simulink model "ps_isop_rail"  (R2026a)
settings: Solver=ode23tb  StopTime=param.sim.simlength  FixedStep=param.glb_time.tc  MaxStep=param.glb_time.tc
values from neighbouring files (symbols this model uses):
  param = struct()    [init_model.m]
libraries: fl_lib x49, nesl_utility x38, full_bridge_ideal_switch x4, single_phase_transformer x4, pi_ctrl x3, full_bridge_diode_rectifier x2, lithium_ion_battery x1, full_bridge_zvs_pwm_modulator x1, discrete_time_low_pass_filter x1
(part 2 of 2)

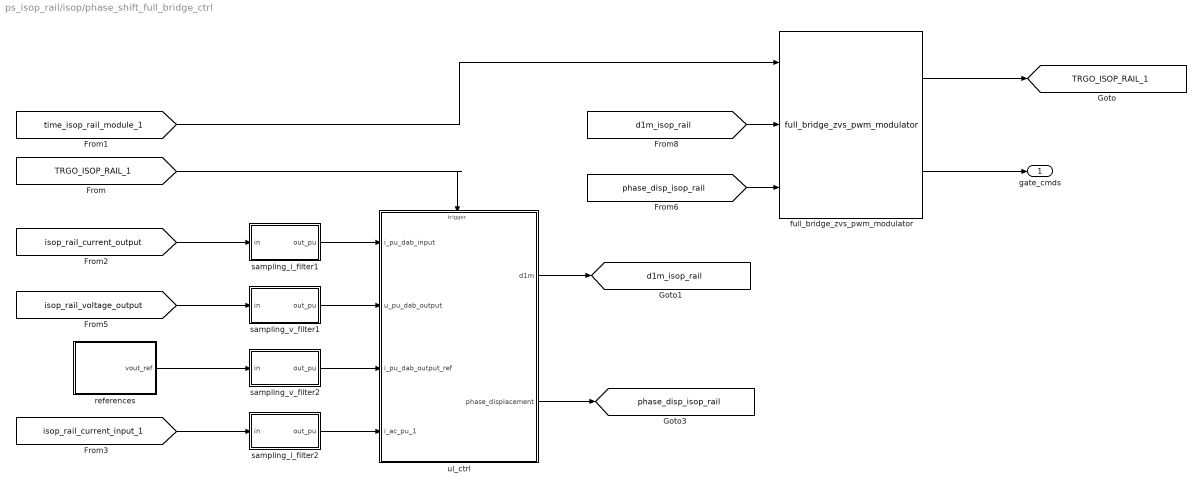
== system ps_isop_rail/isop/phase_shift_full_bridge_ctrl ==
  full_bridge_zvs_pwm_modulator : full_bridge_zvs_pwm_modulator/full_bridge_zvs_pwm_modulator  fPWM_m=param.glb_time.fPWM_ISOP_RAIL  m_up_m=1  m_low_m=0  dead_time_DAB_m=param.glb_time.dead_time_ISOP_RAIL  pos_cmd_gate_m=15  neg_cmd_gate_m=-10  polarity_m=1  tc_m=param.glb_time.tc  max_phase_displacement_m=pi  trgo_double_update_m=param.glb_time.TRGO_ISOP_RAIL_double_update
  references : Subsystem
  sampling_i_filter1 : Subsystem
  sampling_i_filter2 : Subsystem
  sampling_v_filter1 : Subsystem
  sampling_v_filter2 : Subsystem
  ui_ctrl : Subsystem
  gate_cmds : Outport
  tag scope: TRGO_ISOP_RAIL_1=global, d1m_isop_rail=global, phase_disp_isop_rail=global
  wires:
  [isop_rail_voltage_output] -> sampling_v_filter1/1(in)
  [isop_rail_current_output] -> sampling_i_filter1/1(in)
  sampling_i_filter1/1(out_pu) -> ui_ctrl/1(i_pu_dab_input)
  sampling_v_filter1/1(out_pu) -> ui_ctrl/2(u_pu_dab_output)
  sampling_v_filter2/1(out_pu) -> ui_ctrl/3(i_pu_dab_output_ref)
  references/1(vout_ref) -> sampling_v_filter2/1(in)
  full_bridge_zvs_pwm_modulator/2 -> gate_cmds/1
  [time_isop_rail_module_1] -> full_bridge_zvs_pwm_modulator/1
  full_bridge_zvs_pwm_modulator/1 -> [TRGO_ISOP_RAIL_1]
  [TRGO_ISOP_RAIL_1] -> ui_ctrl/Trigger
  [isop_rail_current_input_1] -> sampling_i_filter2/1(in)
  sampling_i_filter2/1(out_pu) -> ui_ctrl/4(i_ac_pu_1)
  ui_ctrl/1(d1m) -> [d1m_isop_rail]
  ui_ctrl/2(phase_displacement) -> [phase_disp_isop_rail]
  [phase_disp_isop_rail] -> full_bridge_zvs_pwm_modulator/3
  [d1m_isop_rail] -> full_bridge_zvs_pwm_modulator/2

== system ps_isop_rail/isop/rectifier_1 ==
  full_bridge_diode_rectifier : full_bridge_diode_rectifier/full_bridge_diode_rectifier  Vf_diode_rectifier=param.diode.rectifier.Vf  Rdon_diode_rectifier=param.diode.rectifier.Rdon  Csnubber=param.diode.rectifier.Csnubber  Rsnubber=param.diode.rectifier.Rsnubber
  uac_2(+) : PMIOPort  Side=Left
  uac_2(-) : PMIOPort  Port=2  Side=Left
  udc_1(+) : PMIOPort  Port=3  Side=Right
  udc_1(-) : PMIOPort  Port=4  Side=Right
  tag scope: diode_bridge_1=global
  wires:
  full_bridge_diode_rectifier/1 -> [diode_bridge_1]
  connections:
  udc_1(-)/RConn1 -- full_bridge_diode_rectifier/RConn2
  full_bridge_diode_rectifier/LConn1 -- uac_2(+)/RConn1
  full_bridge_diode_rectifier/LConn2 -- uac_2(-)/RConn1
  udc_1(+)/RConn1 -- full_bridge_diode_rectifier/RConn1

== system ps_isop_rail/isop/rectifier_2 ==
  full_bridge_diode_rectifier : full_bridge_diode_rectifier/full_bridge_diode_rectifier  Vf_diode_rectifier=param.diode.rectifier.Vf  Rdon_diode_rectifier=param.diode.rectifier.Rdon  Csnubber=param.diode.rectifier.Csnubber  Rsnubber=param.diode.rectifier.Rsnubber
  uac_2(+) : PMIOPort  Side=Left
  uac_2(-) : PMIOPort  Port=2  Side=Left
  udc_2(+) : PMIOPort  Port=3  Side=Right
  udc_2(-) : PMIOPort  Port=4  Side=Right
  tag scope: diode_bridge_2=global
  wires:
  full_bridge_diode_rectifier/1 -> [diode_bridge_2]
  connections:
  udc_2(+)/RConn1 -- full_bridge_diode_rectifier/RConn1
  full_bridge_diode_rectifier/LConn2 -- uac_2(-)/RConn1
  full_bridge_diode_rectifier/LConn1 -- uac_2(+)/RConn1
  udc_2(-)/RConn1 -- full_bridge_diode_rectifier/RConn2

== system ps_isop_rail/isop/fb_iso_mod_1/full_bridge ==
  gate_commands : Inport
  full-bridge_ideal_switch_based : Subsystem
  uac_1(+) : PMIOPort  Side=Left
  uac_1(-) : PMIOPort  Port=2  Side=Left
  Udc(+) : PMIOPort  Port=3  Side=Right
  Udc(-) : PMIOPort  Port=4  Side=Right
  wires:
  gate_commands/1 -> full-bridge_ideal_switch_based/1(gate_commands)
  connections:
  uac_1(-)/RConn1 -- full-bridge_ideal_switch_based/RConn2
  Udc(-)/RConn1 -- full-bridge_ideal_switch_based/LConn2
  Udc(+)/RConn1 -- full-bridge_ideal_switch_based/LConn1
  full-bridge_ideal_switch_based/RConn1 -- uac_1(+)/RConn1

== system ps_isop_rail/isop/fb_iso_mod_1/transformers ==
  Current Sensor1 : fl_lib/Electrical/Electrical Sensors/Current Sensor
  Voltage Sensor1 : fl_lib/Electrical/Electrical Sensors/Voltage Sensor
  i1_transformer : nesl_utility/PS-Simulink Converter  PhysicalDomain=network_engine_domain  SubClassName=ps_output  LeftPortType=input  RightPortType=output  PseudoPeriodic=off  Frequencies=[]  VectorFormat=1-D array  Unit=A  AffineConversion=off
  trafo_1 : Subsystem
  u1_transformer : nesl_utility/PS-Simulink Converter  PhysicalDomain=network_engine_domain  SubClassName=ps_output  LeftPortType=input  RightPortType=output  PseudoPeriodic=off  Frequencies=[]  VectorFormat=1-D array  Unit=V  AffineConversion=on
  uac_1(+) : PMIOPort  Side=Left
  uac_1(-) : PMIOPort  Port=2  Side=Left
  uac_2(+) : PMIOPort  Port=3  Side=Right
  uac_2(-) : PMIOPort  Port=4  Side=Right
  tag scope: i1_trafo_mod_1=global, u1_trafo_mod_1=global
  wires:
  u1_transformer/1 -> [u1_trafo_mod_1]
  i1_transformer/1 -> [i1_trafo_mod_1]
  connections:
  trafo_1/LConn1 -- Current Sensor1/RConn2
  uac_1(-)/RConn1 -- Voltage Sensor1/RConn2 -- trafo_1/LConn2
  trafo_1/RConn1 -- uac_2(+)/RConn1
  trafo_1/RConn2 -- uac_2(-)/RConn1
  Voltage Sensor1/LConn1 -- Current Sensor1/LConn1 -- uac_1(+)/RConn1
  Voltage Sensor1/RConn1 -- u1_transformer/LConn1
  Current Sensor1/RConn1 -- i1_transformer/LConn1

== system ps_isop_rail/isop/fb_iso_mod_2/full_bridge ==
  gate_commands : Inport
  full-bridge_ideal_switch_based : Subsystem
  uac_1(+) : PMIOPort  Side=Left
  uac_1(-) : PMIOPort  Port=2  Side=Left
  Udc(+) : PMIOPort  Port=3  Side=Right
  Udc(-) : PMIOPort  Port=4  Side=Right
  wires:
  gate_commands/1 -> full-bridge_ideal_switch_based/1(gate_commands)
  connections:
  full-bridge_ideal_switch_based/RConn1 -- uac_1(+)/RConn1
  Udc(+)/RConn1 -- full-bridge_ideal_switch_based/LConn1
  Udc(-)/RConn1 -- full-bridge_ideal_switch_based/LConn2
  uac_1(-)/RConn1 -- full-bridge_ideal_switch_based/RConn2

== system ps_isop_rail/isop/fb_iso_mod_2/transformers ==
  Current Sensor1 : fl_lib/Electrical/Electrical Sensors/Current Sensor
  Voltage Sensor1 : fl_lib/Electrical/Electrical Sensors/Voltage Sensor
  i1_transformer : nesl_utility/PS-Simulink Converter  PhysicalDomain=network_engine_domain  SubClassName=ps_output  LeftPortType=input  RightPortType=output  PseudoPeriodic=off  Frequencies=[]  VectorFormat=1-D array  Unit=A  AffineConversion=off
  trafo_1 : Subsystem
  u1_transformer : nesl_utility/PS-Simulink Converter  PhysicalDomain=network_engine_domain  SubClassName=ps_output  LeftPortType=input  RightPortType=output  PseudoPeriodic=off  Frequencies=[]  VectorFormat=1-D array  Unit=V  AffineConversion=on
  uac_1(+) : PMIOPort  Side=Left
  uac_1(-) : PMIOPort  Port=2  Side=Left
  uac_2(+) : PMIOPort  Port=3  Side=Right
  uac_2(-) : PMIOPort  Port=4  Side=Right
  tag scope: i1_trafo_mod_2=global, u1_trafo_mod_2=global
  wires:
  i1_transformer/1 -> [i1_trafo_mod_2]
  u1_transformer/1 -> [u1_trafo_mod_2]
  connections:
  Current Sensor1/RConn1 -- i1_transformer/LConn1
  Voltage Sensor1/RConn1 -- u1_transformer/LConn1
  uac_1(+)/RConn1 -- Current Sensor1/LConn1 -- Voltage Sensor1/LConn1
  trafo_1/RConn2 -- uac_2(-)/RConn1
  trafo_1/RConn1 -- uac_2(+)/RConn1
  trafo_1/LConn2 -- Voltage Sensor1/RConn2 -- uac_1(-)/RConn1
  trafo_1/LConn1 -- Current Sensor1/RConn2

== system ps_isop_rail/isop/fb_iso_mod_3/full_bridge ==
  gate_commands : Inport
  full-bridge_ideal_switch_based : Subsystem
  uac_1(+) : PMIOPort  Side=Left
  uac_1(-) : PMIOPort  Port=2  Side=Left
  Udc(+) : PMIOPort  Port=3  Side=Right
  Udc(-) : PMIOPort  Port=4  Side=Right
  wires:
  gate_commands/1 -> full-bridge_ideal_switch_based/1(gate_commands)
  connections:
  uac_1(-)/RConn1 -- full-bridge_ideal_switch_based/RConn2
  Udc(-)/RConn1 -- full-bridge_ideal_switch_based/LConn2
  Udc(+)/RConn1 -- full-bridge_ideal_switch_based/LConn1
  full-bridge_ideal_switch_based/RConn1 -- uac_1(+)/RConn1

== system ps_isop_rail/isop/fb_iso_mod_3/transformers ==
  Current Sensor1 : fl_lib/Electrical/Electrical Sensors/Current Sensor
  Voltage Sensor1 : fl_lib/Electrical/Electrical Sensors/Voltage Sensor
  i1_transformer : nesl_utility/PS-Simulink Converter  PhysicalDomain=network_engine_domain  SubClassName=ps_output  LeftPortType=input  RightPortType=output  PseudoPeriodic=off  Frequencies=[]  VectorFormat=1-D array  Unit=A  AffineConversion=off
  trafo_1 : Subsystem
  u1_transformer : nesl_utility/PS-Simulink Converter  PhysicalDomain=network_engine_domain  SubClassName=ps_output  LeftPortType=input  RightPortType=output  PseudoPeriodic=off  Frequencies=[]  VectorFormat=1-D array  Unit=V  AffineConversion=on
  uac_1(+) : PMIOPort  Side=Left
  uac_1(-) : PMIOPort  Port=2  Side=Left
  uac_2(+) : PMIOPort  Port=3  Side=Right
  uac_2(-) : PMIOPort  Port=4  Side=Right
  tag scope: i1_trafo_mod_3=global, u1_trafo_mod_3=global
  wires:
  u1_transformer/1 -> [u1_trafo_mod_3]
  i1_transformer/1 -> [i1_trafo_mod_3]
  connections:
  trafo_1/LConn1 -- Current Sensor1/RConn2
  uac_1(-)/RConn1 -- Voltage Sensor1/RConn2 -- trafo_1/LConn2
  trafo_1/RConn1 -- uac_2(+)/RConn1
  trafo_1/RConn2 -- uac_2(-)/RConn1
  Voltage Sensor1/LConn1 -- Current Sensor1/LConn1 -- uac_1(+)/RConn1
  Voltage Sensor1/RConn1 -- u1_transformer/LConn1
  Current Sensor1/RConn1 -- i1_transformer/LConn1

== system ps_isop_rail/isop/fb_iso_mod_4/full_bridge ==
  gate_commands : Inport
  full-bridge_ideal_switch_based : Subsystem
  uac_1(+) : PMIOPort  Side=Left
  uac_1(-) : PMIOPort  Port=2  Side=Left
  Udc(+) : PMIOPort  Port=3  Side=Right
  Udc(-) : PMIOPort  Port=4  Side=Right
  wires:
  gate_commands/1 -> full-bridge_ideal_switch_based/1(gate_commands)
  connections:
  full-bridge_ideal_switch_based/RConn1 -- uac_1(+)/RConn1
  Udc(+)/RConn1 -- full-bridge_ideal_switch_based/LConn1
  Udc(-)/RConn1 -- full-bridge_ideal_switch_based/LConn2
  uac_1(-)/RConn1 -- full-bridge_ideal_switch_based/RConn2

== system ps_isop_rail/isop/fb_iso_mod_4/transformers ==
  Current Sensor1 : fl_lib/Electrical/Electrical Sensors/Current Sensor
  Voltage Sensor1 : fl_lib/Electrical/Electrical Sensors/Voltage Sensor
  i1_transformer : nesl_utility/PS-Simulink Converter  PhysicalDomain=network_engine_domain  SubClassName=ps_output  LeftPortType=input  RightPortType=output  PseudoPeriodic=off  Frequencies=[]  VectorFormat=1-D array  Unit=A  AffineConversion=off
  trafo_1 : Subsystem
  u1_transformer : nesl_utility/PS-Simulink Converter  PhysicalDomain=network_engine_domain  SubClassName=ps_output  LeftPortType=input  RightPortType=output  PseudoPeriodic=off  Frequencies=[]  VectorFormat=1-D array  Unit=V  AffineConversion=on
  uac_1(+) : PMIOPort  Side=Left
  uac_1(-) : PMIOPort  Port=2  Side=Left
  uac_2(+) : PMIOPort  Port=3  Side=Right
  uac_2(-) : PMIOPort  Port=4  Side=Right
  tag scope: i1_trafo_mod_4=global, u1_trafo_mod_4=global
  wires:
  i1_transformer/1 -> [i1_trafo_mod_4]
  u1_transformer/1 -> [u1_trafo_mod_4]
  connections:
  Current Sensor1/RConn1 -- i1_transformer/LConn1
  Voltage Sensor1/RConn1 -- u1_transformer/LConn1
  uac_1(+)/RConn1 -- Current Sensor1/LConn1 -- Voltage Sensor1/LConn1
  trafo_1/RConn2 -- uac_2(-)/RConn1
  trafo_1/RConn1 -- uac_2(+)/RConn1
  trafo_1/LConn2 -- Voltage Sensor1/RConn2 -- uac_1(-)/RConn1
  trafo_1/LConn1 -- Current Sensor1/RConn2

== system ps_isop_rail/isop/phase_shift_full_bridge_ctrl/references ==
  Rate Limiter : RateLimiter  RisingSlewLimit=param.isop_rail.hw.idc2_nom*10  FallingSlewLimit=-param.isop_rail.hw.idc2_nom*10  SampleTimeMode=inherited
  Vout_dc_nom : Step  Time=0.025  FinalValue=param.isop_rail.hw.idc2_nom  SampleTime=0
  vout_ref : Outport
  wires:
  Rate Limiter/1 -> vout_ref/1
  Vout_dc_nom/1 -> Rate Limiter/1

== system ps_isop_rail/isop/phase_shift_full_bridge_ctrl/sampling_i_filter1 ==
  in : Inport
  1/Ti3 : Gain  Gain=1/param.isop_rail.hw.idc2_bez  OutDataTypeStr=double  SaturateOnIntegerOverflow=on  ParamDataTypeStr=Inherit: Same as input
  out_pu : Outport
  wires:
  in/1 -> 1/Ti3/1
  1/Ti3/1 -> out_pu/1

== system ps_isop_rail/isop/phase_shift_full_bridge_ctrl/sampling_i_filter2 ==
  in : Inport
  1/Ti3 : Gain  Gain=1/param.isop_rail.hw.idc1_bez  OutDataTypeStr=double  SaturateOnIntegerOverflow=on  ParamDataTypeStr=Inherit: Same as input
  out_pu : Outport
  wires:
  1/Ti3/1 -> out_pu/1
  in/1 -> 1/Ti3/1

== system ps_isop_rail/isop/phase_shift_full_bridge_ctrl/sampling_v_filter1 ==
  in : Inport
  1/Ti3 : Gain  Gain=1/param.isop_rail.hw.udc2_bez  OutDataTypeStr=double  SaturateOnIntegerOverflow=on  ParamDataTypeStr=Inherit: Same as input
  out_pu : Outport
  wires:
  in/1 -> 1/Ti3/1
  1/Ti3/1 -> out_pu/1

== system ps_isop_rail/isop/phase_shift_full_bridge_ctrl/sampling_v_filter2 ==
  in : Inport
  1/Ti3 : Gain  Gain=1/param.isop_rail.hw.idc2_nom  OutDataTypeStr=double  SaturateOnIntegerOverflow=on  ParamDataTypeStr=Inherit: Same as input
  Saturation : Saturate  UpperLimit=1  LowerLimit=0  OutDataTypeStr=double
  out_pu : Outport
  wires:
  in/1 -> 1/Ti3/1
  1/Ti3/1 -> Saturation/1
  Saturation/1 -> out_pu/1

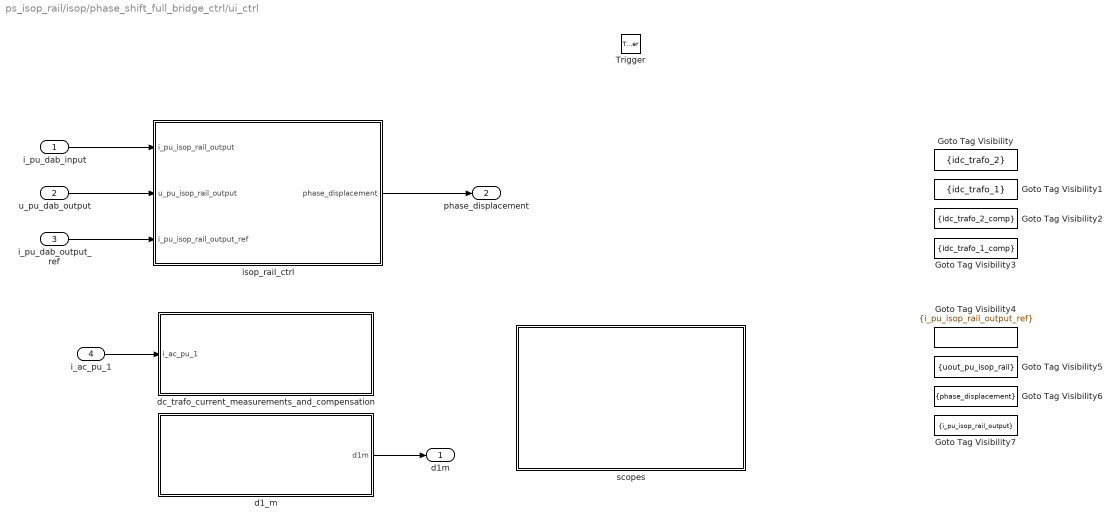
== system ps_isop_rail/isop/phase_shift_full_bridge_ctrl/ui_ctrl ==
  i_pu_dab_input : Inport
  u_pu_dab_output : Inport  Port=2
  i_pu_dab_output_ref : Inport  Port=3
  i_ac_pu_1 : Inport  Port=4
  Trigger : TriggerPort  VariantControl=(inherit)  PortDimensions=1
  Goto Tag Visibility : GotoTagVisibility  GotoTag=idc_trafo_2
  Goto Tag Visibility1 : GotoTagVisibility  GotoTag=idc_trafo_1
  Goto Tag Visibility2 : GotoTagVisibility  GotoTag=idc_trafo_2_comp
  Goto Tag Visibility3 : GotoTagVisibility  GotoTag=idc_trafo_1_comp
  Goto Tag Visibility4 : GotoTagVisibility  GotoTag=i_pu_isop_rail_output_ref
  Goto Tag Visibility5 : GotoTagVisibility  GotoTag=uout_pu_isop_rail
  Goto Tag Visibility6 : GotoTagVisibility  GotoTag=phase_displacement
  Goto Tag Visibility7 : GotoTagVisibility  GotoTag=i_pu_isop_rail_output
  d1_m : Subsystem
  dc_trafo_current_measurements_and_compensation : Subsystem
  isop_rail_ctrl : Subsystem
  scopes : Subsystem
  d1m : Outport
  phase_displacement : Outport  Port=2
  wires:
  i_pu_dab_input/1 -> isop_rail_ctrl/1(i_pu_isop_rail_output)
  u_pu_dab_output/1 -> isop_rail_ctrl/2(u_pu_isop_rail_output)
  i_pu_dab_output_ref/1 -> isop_rail_ctrl/3(i_pu_isop_rail_output_ref)
  i_ac_pu_1/1 -> dc_trafo_current_measurements_and_compensation/1(i_ac_pu_1)
  d1_m/1(d1m) -> d1m/1
  isop_rail_ctrl/1(phase_displacement) -> phase_displacement/1

== system ps_isop_rail/isop/fb_iso_mod_1/full_bridge/full-bridge_ideal_switch_based ==
  gate_commands : Inport
  full-bridge ideal switch based : full_bridge_ideal_switch/full-bridge ideal switch based  Rds_on=param.isop_rail.ideal_switch.Rds_on  Vdon_diode=param.isop_rail.ideal_switch.Vdon_diode  Rdon_diode=param.isop_rail.ideal_switch.Rdon_diode  Csnubber=param.isop_rail.ideal_switch.Csnubber  Rsnubber=param.isop_rail.ideal_switch.Rsnubber  Vth=param.isop_rail.ideal_switch.Vth
  udc(+) : PMIOPort  Side=Left
  uac(+) : PMIOPort  Port=2  Side=Right
  udc(-) : PMIOPort  Port=3  Side=Left
  uac(-) : PMIOPort  Port=4  Side=Right
  wires:
  gate_commands/1 -> full-bridge ideal switch based/1
  connections:
  full-bridge ideal switch based/RConn2 -- uac(-)/RConn1
  full-bridge ideal switch based/LConn2 -- udc(-)/RConn1
  full-bridge ideal switch based/RConn1 -- uac(+)/RConn1
  full-bridge ideal switch based/LConn1 -- udc(+)/RConn1

== system ps_isop_rail/isop/fb_iso_mod_1/transformers/trafo_1 ==
  Current Sensor : fl_lib/Electrical/Electrical Sensors/Current Sensor
  Voltage Sensor3 : fl_lib/Electrical/Electrical Sensors/Voltage Sensor
  i2_transformer : nesl_utility/PS-Simulink Converter  PhysicalDomain=network_engine_domain  SubClassName=ps_output  LeftPortType=input  RightPortType=output  PseudoPeriodic=off  Frequencies=[]  VectorFormat=1-D array  Unit=A  AffineConversion=off
  single_phase_transformer : single_phase_transformer/single_phase_transformer  lm_trafo=param.isop_rail.hw.Lm  m1=param.isop_rail.hw.n1  m2=param.isop_rail.hw.n2  rd1_trafo=param.isop_rail.hw.Rs1  rd2_trafo=param.isop_rail.hw.Rs2  ld1_trafo=param.isop_rail.hw.Ld1  ld2_trafo=param.isop_rail.hw.Ld2  rfe_trafo=param.isop_rail.hw.Rfe  length_core=param.isop_rail.hw.core_length  mu0=param.isop_rail.hw.mu0  mur=param.isop_rail.hw.core_mur
  single_phase_transformer - scope : Scope
      settings: ActiveDisplayYMinimum=-18.928487063481988  ActiveDisplayYMaximum=20.382917044296853  DataLoggingVariableName=ScopeData21
  u2_transformer : nesl_utility/PS-Simulink Converter  PhysicalDomain=network_engine_domain  SubClassName=ps_output  LeftPortType=input  RightPortType=output  PseudoPeriodic=off  Frequencies=[]  VectorFormat=1-D array  Unit=V  AffineConversion=on
  uac_1(+) : PMIOPort  Side=Left
  uac_1(-) : PMIOPort  Port=2  Side=Left
  uac_2(+) : PMIOPort  Port=3  Side=Right
  uac_2(-) : PMIOPort  Port=4  Side=Right
  tag scope: i2_trafo_mod_1=global, u2_trafo_mod_1=global
  wires:
  single_phase_transformer/1 -> single_phase_transformer - scope/1
  u2_transformer/1 -> [u2_trafo_mod_1]
  i2_transformer/1 -> [i2_trafo_mod_1]
  connections:
  single_phase_transformer/LConn2 -- uac_1(-)/RConn1
  uac_2(-)/RConn1 -- single_phase_transformer/RConn2 -- Voltage Sensor3/RConn2
  Voltage Sensor3/RConn1 -- u2_transformer/LConn1
  single_phase_transformer/LConn1 -- uac_1(+)/RConn1
  Current Sensor/LConn1 -- Voltage Sensor3/LConn1 -- single_phase_transformer/RConn1
  Current Sensor/RConn2 -- uac_2(+)/RConn1
  Current Sensor/RConn1 -- i2_transformer/LConn1

== system ps_isop_rail/isop/fb_iso_mod_2/full_bridge/full-bridge_ideal_switch_based ==
  gate_commands : Inport
  full-bridge ideal switch based : full_bridge_ideal_switch/full-bridge ideal switch based  Rds_on=param.isop_rail.ideal_switch.Rds_on  Vdon_diode=param.isop_rail.ideal_switch.Vdon_diode  Rdon_diode=param.isop_rail.ideal_switch.Rdon_diode  Csnubber=param.isop_rail.ideal_switch.Csnubber  Rsnubber=param.isop_rail.ideal_switch.Rsnubber  Vth=param.isop_rail.ideal_switch.Vth
  udc(+) : PMIOPort  Side=Left
  uac(+) : PMIOPort  Port=2  Side=Right
  udc(-) : PMIOPort  Port=3  Side=Left
  uac(-) : PMIOPort  Port=4  Side=Right
  wires:
  gate_commands/1 -> full-bridge ideal switch based/1
  connections:
  udc(+)/RConn1 -- full-bridge ideal switch based/LConn1
  full-bridge ideal switch based/RConn1 -- uac(+)/RConn1
  udc(-)/RConn1 -- full-bridge ideal switch based/LConn2
  uac(-)/RConn1 -- full-bridge ideal switch based/RConn2

== system ps_isop_rail/isop/fb_iso_mod_2/transformers/trafo_1 ==
  Current Sensor : fl_lib/Electrical/Electrical Sensors/Current Sensor
  Voltage Sensor3 : fl_lib/Electrical/Electrical Sensors/Voltage Sensor
  i2_transformer : nesl_utility/PS-Simulink Converter  PhysicalDomain=network_engine_domain  SubClassName=ps_output  LeftPortType=input  RightPortType=output  PseudoPeriodic=off  Frequencies=[]  VectorFormat=1-D array  Unit=A  AffineConversion=off
  single_phase_transformer : single_phase_transformer/single_phase_transformer  lm_trafo=param.isop_rail.hw.Lm  m1=param.isop_rail.hw.n1  m2=param.isop_rail.hw.n2  rd1_trafo=param.isop_rail.hw.Rs1  rd2_trafo=param.isop_rail.hw.Rs2  ld1_trafo=param.isop_rail.hw.Ld1  ld2_trafo=param.isop_rail.hw.Ld2  rfe_trafo=param.isop_rail.hw.Rfe  length_core=param.isop_rail.hw.core_length  mu0=param.isop_rail.hw.mu0  mur=param.isop_rail.hw.core_mur
  single_phase_transformer - scope : Scope
      settings: ActiveDisplayYMinimum=-18.928487063481988  ActiveDisplayYMaximum=20.382917044296853  DataLoggingVariableName=ScopeData21
  u2_transformer : nesl_utility/PS-Simulink Converter  PhysicalDomain=network_engine_domain  SubClassName=ps_output  LeftPortType=input  RightPortType=output  PseudoPeriodic=off  Frequencies=[]  VectorFormat=1-D array  Unit=V  AffineConversion=on
  uac_1(+) : PMIOPort  Side=Left
  uac_1(-) : PMIOPort  Port=2  Side=Left
  uac_2(+) : PMIOPort  Port=3  Side=Right
  uac_2(-) : PMIOPort  Port=4  Side=Right
  tag scope: i2_trafo_mod_2=global, u2_trafo_mod_2=global
  wires:
  i2_transformer/1 -> [i2_trafo_mod_2]
  u2_transformer/1 -> [u2_trafo_mod_2]
  single_phase_transformer/1 -> single_phase_transformer - scope/1
  connections:
  Current Sensor/RConn1 -- i2_transformer/LConn1
  Current Sensor/RConn2 -- uac_2(+)/RConn1
  single_phase_transformer/RConn1 -- Voltage Sensor3/LConn1 -- Current Sensor/LConn1
  single_phase_transformer/LConn1 -- uac_1(+)/RConn1
  Voltage Sensor3/RConn1 -- u2_transformer/LConn1
  Voltage Sensor3/RConn2 -- single_phase_transformer/RConn2 -- uac_2(-)/RConn1
  single_phase_transformer/LConn2 -- uac_1(-)/RConn1

== system ps_isop_rail/isop/fb_iso_mod_3/full_bridge/full-bridge_ideal_switch_based ==
  gate_commands : Inport
  full-bridge ideal switch based : full_bridge_ideal_switch/full-bridge ideal switch based  Rds_on=param.isop_rail.ideal_switch.Rds_on  Vdon_diode=param.isop_rail.ideal_switch.Vdon_diode  Rdon_diode=param.isop_rail.ideal_switch.Rdon_diode  Csnubber=param.isop_rail.ideal_switch.Csnubber  Rsnubber=param.isop_rail.ideal_switch.Rsnubber  Vth=param.isop_rail.ideal_switch.Vth
  udc(+) : PMIOPort  Side=Left
  uac(+) : PMIOPort  Port=2  Side=Right
  udc(-) : PMIOPort  Port=3  Side=Left
  uac(-) : PMIOPort  Port=4  Side=Right
  wires:
  gate_commands/1 -> full-bridge ideal switch based/1
  connections:
  full-bridge ideal switch based/RConn2 -- uac(-)/RConn1
  full-bridge ideal switch based/LConn2 -- udc(-)/RConn1
  full-bridge ideal switch based/RConn1 -- uac(+)/RConn1
  full-bridge ideal switch based/LConn1 -- udc(+)/RConn1

== system ps_isop_rail/isop/fb_iso_mod_3/transformers/trafo_1 ==
  Current Sensor : fl_lib/Electrical/Electrical Sensors/Current Sensor
  Voltage Sensor3 : fl_lib/Electrical/Electrical Sensors/Voltage Sensor
  i2_transformer : nesl_utility/PS-Simulink Converter  PhysicalDomain=network_engine_domain  SubClassName=ps_output  LeftPortType=input  RightPortType=output  PseudoPeriodic=off  Frequencies=[]  VectorFormat=1-D array  Unit=A  AffineConversion=off
  single_phase_transformer : single_phase_transformer/single_phase_transformer  lm_trafo=param.isop_rail.hw.Lm  m1=param.isop_rail.hw.n1  m2=param.isop_rail.hw.n2  rd1_trafo=param.isop_rail.hw.Rs1  rd2_trafo=param.isop_rail.hw.Rs2  ld1_trafo=param.isop_rail.hw.Ld1  ld2_trafo=param.isop_rail.hw.Ld2  rfe_trafo=param.isop_rail.hw.Rfe  length_core=param.isop_rail.hw.core_length  mu0=param.isop_rail.hw.mu0  mur=param.isop_rail.hw.core_mur
  single_phase_transformer - scope : Scope
      settings: ActiveDisplayYMinimum=-18.928487063481988  ActiveDisplayYMaximum=20.382917044296853  DataLoggingVariableName=ScopeData21
  u2_transformer : nesl_utility/PS-Simulink Converter  PhysicalDomain=network_engine_domain  SubClassName=ps_output  LeftPortType=input  RightPortType=output  PseudoPeriodic=off  Frequencies=[]  VectorFormat=1-D array  Unit=V  AffineConversion=on
  uac_1(+) : PMIOPort  Side=Left
  uac_1(-) : PMIOPort  Port=2  Side=Left
  uac_2(+) : PMIOPort  Port=3  Side=Right
  uac_2(-) : PMIOPort  Port=4  Side=Right
  tag scope: i2_trafo_mod_3=global, u2_trafo_mod_3=global
  wires:
  single_phase_transformer/1 -> single_phase_transformer - scope/1
  u2_transformer/1 -> [u2_trafo_mod_3]
  i2_transformer/1 -> [i2_trafo_mod_3]
  connections:
  single_phase_transformer/LConn2 -- uac_1(-)/RConn1
  uac_2(-)/RConn1 -- single_phase_transformer/RConn2 -- Voltage Sensor3/RConn2
  Voltage Sensor3/RConn1 -- u2_transformer/LConn1
  single_phase_transformer/LConn1 -- uac_1(+)/RConn1
  Current Sensor/LConn1 -- Voltage Sensor3/LConn1 -- single_phase_transformer/RConn1
  Current Sensor/RConn2 -- uac_2(+)/RConn1
  Current Sensor/RConn1 -- i2_transformer/LConn1

== system ps_isop_rail/isop/fb_iso_mod_4/full_bridge/full-bridge_ideal_switch_based ==
  gate_commands : Inport
  full-bridge ideal switch based : full_bridge_ideal_switch/full-bridge ideal switch based  Rds_on=param.isop_rail.ideal_switch.Rds_on  Vdon_diode=param.isop_rail.ideal_switch.Vdon_diode  Rdon_diode=param.isop_rail.ideal_switch.Rdon_diode  Csnubber=param.isop_rail.ideal_switch.Csnubber  Rsnubber=param.isop_rail.ideal_switch.Rsnubber  Vth=param.isop_rail.ideal_switch.Vth
  udc(+) : PMIOPort  Side=Left
  uac(+) : PMIOPort  Port=2  Side=Right
  udc(-) : PMIOPort  Port=3  Side=Left
  uac(-) : PMIOPort  Port=4  Side=Right
  wires:
  gate_commands/1 -> full-bridge ideal switch based/1
  connections:
  full-bridge ideal switch based/LConn1 -- udc(+)/RConn1
  full-bridge ideal switch based/RConn1 -- uac(+)/RConn1
  full-bridge ideal switch based/LConn2 -- udc(-)/RConn1
  full-bridge ideal switch based/RConn2 -- uac(-)/RConn1

== system ps_isop_rail/isop/fb_iso_mod_4/transformers/trafo_1 ==
  Current Sensor : fl_lib/Electrical/Electrical Sensors/Current Sensor
  Voltage Sensor3 : fl_lib/Electrical/Electrical Sensors/Voltage Sensor
  i2_transformer : nesl_utility/PS-Simulink Converter  PhysicalDomain=network_engine_domain  SubClassName=ps_output  LeftPortType=input  RightPortType=output  PseudoPeriodic=off  Frequencies=[]  VectorFormat=1-D array  Unit=A  AffineConversion=off
  single_phase_transformer : single_phase_transformer/single_phase_transformer  lm_trafo=param.isop_rail.hw.Lm  m1=param.isop_rail.hw.n1  m2=param.isop_rail.hw.n2  rd1_trafo=param.isop_rail.hw.Rs1  rd2_trafo=param.isop_rail.hw.Rs2  ld1_trafo=param.isop_rail.hw.Ld1  ld2_trafo=param.isop_rail.hw.Ld2  rfe_trafo=param.isop_rail.hw.Rfe  length_core=param.isop_rail.hw.core_length  mu0=param.isop_rail.hw.mu0  mur=param.isop_rail.hw.core_mur
  single_phase_transformer - scope : Scope
      settings: ActiveDisplayYMinimum=-18.928487063481988  ActiveDisplayYMaximum=20.382917044296853  DataLoggingVariableName=ScopeData21
  u2_transformer : nesl_utility/PS-Simulink Converter  PhysicalDomain=network_engine_domain  SubClassName=ps_output  LeftPortType=input  RightPortType=output  PseudoPeriodic=off  Frequencies=[]  VectorFormat=1-D array  Unit=V  AffineConversion=on
  uac_1(+) : PMIOPort  Side=Left
  uac_1(-) : PMIOPort  Port=2  Side=Left
  uac_2(+) : PMIOPort  Port=3  Side=Right
  uac_2(-) : PMIOPort  Port=4  Side=Right
  tag scope: i2_trafo_mod_4=global, u2_trafo_mod_4=global
  wires:
  i2_transformer/1 -> [i2_trafo_mod_4]
  u2_transformer/1 -> [u2_trafo_mod_4]
  single_phase_transformer/1 -> single_phase_transformer - scope/1
  connections:
  Current Sensor/RConn1 -- i2_transformer/LConn1
  Current Sensor/RConn2 -- uac_2(+)/RConn1
  single_phase_transformer/RConn1 -- Voltage Sensor3/LConn1 -- Current Sensor/LConn1
  single_phase_transformer/LConn1 -- uac_1(+)/RConn1
  Voltage Sensor3/RConn1 -- u2_transformer/LConn1
  Voltage Sensor3/RConn2 -- single_phase_transformer/RConn2 -- uac_2(-)/RConn1
  single_phase_transformer/LConn2 -- uac_1(-)/RConn1

== system ps_isop_rail/isop/phase_shift_full_bridge_ctrl/ui_ctrl/d1_m ==
  Constant : Constant  Value=0.5
  Sum : Sum  Inputs=|++
  d1m : Outport
  wires:
  Constant/1 -> Sum/1
  Sum/1 -> d1m/1

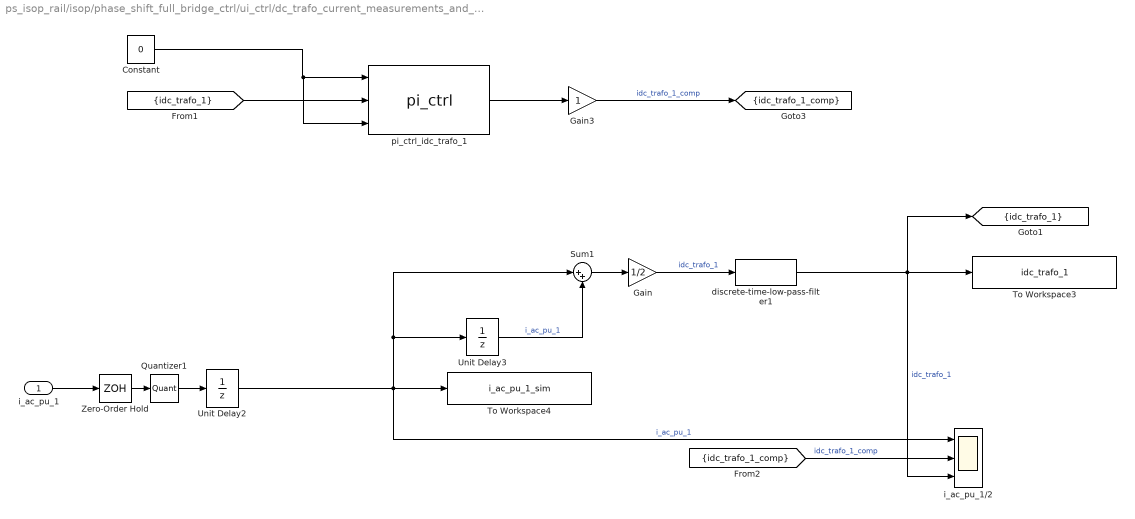
== system ps_isop_rail/isop/phase_shift_full_bridge_ctrl/ui_ctrl/dc_trafo_current_measurements_and_compensation ==
  i_ac_pu_1 : Inport
  Constant : Constant  Value=0
  Gain : Gain  Gain=1/2
  Gain3 : Gain
  Quantizer1 : Quantizer  QuantizationInterval=param.meas.adc12_quantization
  Sum1 : Sum  Inputs=|++
  To Workspace3 : ToWorkspace  VariableName=idc_trafo_1  SampleTime=-1
      settings: MaxDataPoints=param.glb_time.Ns_dab
  To Workspace4 : ToWorkspace  VariableName=i_ac_pu_1_sim  SampleTime=-1
      settings: MaxDataPoints=param.glb_time.Ns_dab
  Unit Delay2 : UnitDelay  SampleTime=-1
  Unit Delay3 : UnitDelay  SampleTime=-1
  Zero-Order Hold : ZeroOrderHold  SampleTime=-1
  discrete-time-low-pass-filter1 : discrete_time_low_pass_filter/discrete-time-low-pass-filter  tau=param.isop_rail.ctrl.tau_idc_trafo  ts=param.glb_time.ts_dab
  i_ac_pu_1/2 : Scope  NumInputPorts=3
      settings: ActiveDisplayYMinimum=-0.044677734374999993  ActiveDisplayYMaximum=0.402099609375  DataLoggingVariableName=ScopeData14
  pi_ctrl_idc_trafo_1 : pi_ctrl/pi_ctrl  kp=param.isop_rail.ctrl.kp_idc_trafo  ki=param.isop_rail.ctrl.ki_idc_trafo  ts=param.glb_time.ts_dab  lim_up=param.isop_rail.ctrl.lim_idc_trafo  lim_down=-param.isop_rail.ctrl.lim_idc_trafo
  tag scope: idc_trafo_1=scoped, idc_trafo_1_comp=scoped
  wires:
  i_ac_pu_1/1 -> Zero-Order Hold/1
  Quantizer1/1 -> Unit Delay2/1
  Unit Delay2/1 -> Sum1/1, Unit Delay3/1, i_ac_pu_1/2/1, To Workspace4/1  "i_ac_pu_1"
  Zero-Order Hold/1 -> Quantizer1/1
  Unit Delay3/1 -> Sum1/2  "i_ac_pu_1"
  Sum1/1 -> Gain/1
  Gain/1 -> discrete-time-low-pass-filter1/1  "idc_trafo_1"
  discrete-time-low-pass-filter1/1 -> To Workspace3/1, [idc_trafo_1], i_ac_pu_1/2/3  "idc_trafo_1"
  [idc_trafo_1] -> pi_ctrl_idc_trafo_1/2
  Constant/1 -> pi_ctrl_idc_trafo_1/3, pi_ctrl_idc_trafo_1/1
  pi_ctrl_idc_trafo_1/1 -> Gain3/1
  Gain3/1 -> [idc_trafo_1_comp]  "idc_trafo_1_comp"
  [idc_trafo_1_comp] -> i_ac_pu_1/2/2  "idc_trafo_1_comp"

== system ps_isop_rail/isop/phase_shift_full_bridge_ctrl/ui_ctrl/isop_rail_ctrl ==
  i_pu_isop_rail_output : Inport
  u_pu_isop_rail_output : Inport  Port=2
  i_pu_isop_rail_output_ref : Inport  Port=3
  Constant : Constant  Value=param.isop_rail.ctrl.udc_ref
  Quantizer1 : Quantizer  QuantizationInterval=param.meas.adc12_quantization
  Quantizer2 : Quantizer  QuantizationInterval=param.meas.adc12_quantization
  Unit Delay2 : UnitDelay  SampleTime=-1
  Unit Delay3 : UnitDelay  SampleTime=-1
  current control : Subsystem
  voltage control : Subsystem
  phase_displacement : Outport
  tag scope: i_pu_isop_rail_output=scoped, i_pu_isop_rail_output_ref=scoped, phase_displacement=scoped, uout_pu_isop_rail=scoped
  wires:
  i_pu_isop_rail_output_ref/1 -> [i_pu_isop_rail_output_ref], current control/1(iout_ref)  "iout_ref"
  i_pu_isop_rail_output/1 -> Quantizer2/1
  Unit Delay3/1 -> current control/2(iout), [i_pu_isop_rail_output]
  Unit Delay2/1 -> [uout_pu_isop_rail]
  u_pu_isop_rail_output/1 -> Quantizer1/1
  Quantizer1/1 -> Unit Delay2/1
  Quantizer2/1 -> Unit Delay3/1
  voltage control/1(u_ctrl_out) -> [phase_displacement], phase_displacement/1
  Constant/1 -> voltage control/1(uout_ref)
  [uout_pu_isop_rail] -> voltage control/2(uout)

== system ps_isop_rail/isop/phase_shift_full_bridge_ctrl/ui_ctrl/scopes ==
  Bus Creator : BusCreator  Inputs=2
  Bus Creator1 : BusCreator  Inputs=2
  From7 : From  Commented=on  GotoTag=uout_ref_pu_isop_rail
  psfbc-tracking : Scope  NumInputPorts=2
      settings: ActiveDisplayYMinimum=-0.7264395439314022  ActiveDisplayYMaximum=2.2614067014075516  DataLoggingVariableName=ScopeData7
  u_ctrl_out_psfbc/i_ctrl_out_psfbc : Scope  NumInputPorts=2
      settings: ActiveDisplayYMinimum=-0.12499999999999997  ActiveDisplayYMaximum=1.125
  wires:
  Bus Creator1/1 -> psfbc-tracking/2
  Bus Creator/1 -> psfbc-tracking/1
  [phase_displacement] -> u_ctrl_out_psfbc/i_ctrl_out_psfbc/2  "i_ctrl_out_psfbc"
  [i_pu_isop_rail_output] -> Bus Creator1/2  "i_in_pu_psfbc"
  From7/1 -> Bus Creator/1  "uout_ref_pu_psfbc"
  [i_pu_isop_rail_output_ref] -> u_ctrl_out_psfbc/i_ctrl_out_psfbc/1  "u_ctrl_out_psfbc"
  [i_pu_isop_rail_output_ref] -> Bus Creator1/1  "u_ctrl_out_psfbc"
  [uout_pu_isop_rail] -> Bus Creator/2  "uout_pu_psfbc"

== system ps_isop_rail/isop/phase_shift_full_bridge_ctrl/ui_ctrl/isop_rail_ctrl/current control ==
  iout_ref : Inport
  iout : Inport  Port=2
  Gain : Gain  Gain=0
  i_out_isop_rail_tracking : Scope  NumInputPorts=3
      settings: ActiveDisplayYMinimum=-0.12499999999999997  ActiveDisplayYMaximum=1.125  DataLoggingVariableName=ScopeData12
  pi_ctrl : pi_ctrl/pi_ctrl  kp=param.isop_rail.ctrl.kp_idc  ki=param.isop_rail.ctrl.ki_idc  ts=param.glb_time.ts_isop_rail  lim_up=1  lim_down=0
  i_ctrl_out : Outport
  wires:
  iout_ref/1 -> pi_ctrl/1, i_out_isop_rail_tracking/1, Gain/1  "i_out_dab_ref"
  iout/1 -> pi_ctrl/2, i_out_isop_rail_tracking/2  "i_out_dab"
  pi_ctrl/1 -> i_ctrl_out/1, i_out_isop_rail_tracking/3  "i_ctrl_out"
  Gain/1 -> pi_ctrl/3

== system ps_isop_rail/isop/phase_shift_full_bridge_ctrl/ui_ctrl/isop_rail_ctrl/voltage control ==
  uout_ref : Inport
  uout : Inport  Port=2
  Gain : Gain  Gain=0
  pi_ctrl : pi_ctrl/pi_ctrl  kp=param.isop_rail.ctrl.kp_udc  ki=param.isop_rail.ctrl.ki_udc  ts=param.glb_time.ts_isop_rail  lim_up=1  lim_down=0
  u_out_isop_rail_tracking : Scope  NumInputPorts=3
      settings: ActiveDisplayYMinimum=-0.12499999999999997  ActiveDisplayYMaximum=1.125  DataLoggingVariableName=ScopeData12
  u_ctrl_out : Outport
  wires:
  Gain/1 -> pi_ctrl/3
  pi_ctrl/1 -> u_out_isop_rail_tracking/3, u_ctrl_out/1  "ctrl_out"
  uout/1 -> u_out_isop_rail_tracking/2, pi_ctrl/2  "u_out_isop_rail"
  uout_ref/1 -> Gain/1, u_out_isop_rail_tracking/1, pi_ctrl/1  "u_out_isop_rail_ref"
